simulink model "ref_mass_spring_damper"  (R2026a)
settings: Solver=ode45  StopTime=10  FixedStep=1e-3  MaxStep=1e-2  RelTol=1e-10  AbsTol=1e-12
settings Model: Creator=djangovanderplas  LastModifiedBy=djangovanderplas
settings DataIOCC: OutputOption=SpecifiedOutputTimes  OutputTimes=0:1e-3:10

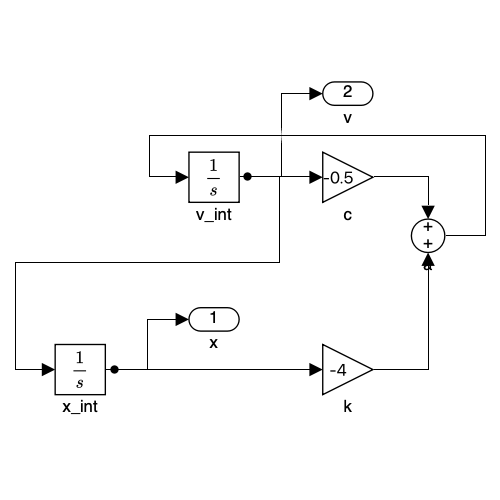
[thumbnail: Simulink's stored preview of the top-level diagram]
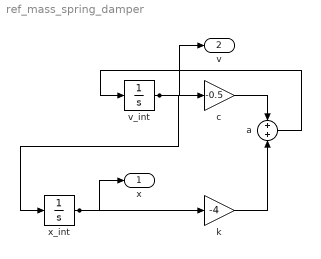
== system ref_mass_spring_damper ==
  a : Sum
  c : Gain  Gain=-0.5
  k : Gain  Gain=-4
  v_int : Integrator
  x_int : Integrator  InitialCondition=1
  x : Outport
  v : Outport  Port=2
  wires:
  a/1 -> v_int/1
  k/1 -> a/2
  c/1 -> a/1
  v_int/1 -> v/1, c/1, x_int/1
  x_int/1 -> x/1, k/1
